simulink library "Batteries"  (R2025b)
settings: Solver=VariableStepAuto  StartTime=0.0  StopTime=10.0  RelTol=1e-3
undefined symbols (not defined in the file or in its folder): battery_builder_rtmsupport, gcbh
libraries: Batteries_lib x12
(part 1 of 2)
settings Model: Creator=Ashwin VJ  LastModifiedBy=Ashwin VJ

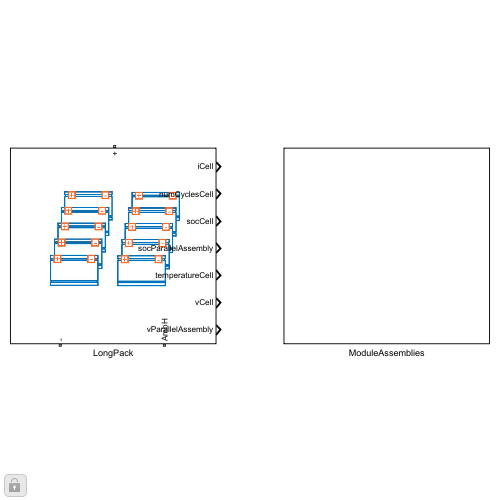
[thumbnail: Simulink's stored preview of the top-level diagram]
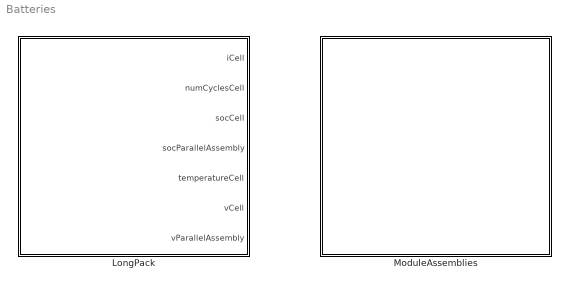
== system Batteries ==
  LongPack : Subsystem  LoadFcn=battery_builder_rtmsupport('loadfcn',gcbh);
      settings: CopyFcn=battery_builder_rtmsupport('copyfcn',gcbh);  PreCopyFcn=battery_builder_rtmsupport('precopyfcn',gcbh);  PreDeleteFcn=battery_builder_rtmsupport('predeletefcn',gcbh);  PortSchema="{\"entries\":[{\"content\":{\"sides\":[{\"content\":{\"connectorIds\":[\"LConn1\"]},\"type\":\"ConnectorPlacement.EquallySpacedRectSide\",\"uuid\":\"4fe37960-74fc-413e-9859-48e6f871084a\"},{\"content\":{\"connectorIds\":[\"RConn1\",\"RConn2\"],\"side\":\"RIGHT\"},\"type\":\"ConnectorPlacement.EquallySpacedRectSide\",\"uuid\":\"59d8cb7e-b3c6-46ea-9337-4df7c2d713cd\"},{\"content\":{\"side\":\"TOP\"},\"type\":\"ConnectorPlacement.EquallySpacedRectSide\",\"uuid\":\"862fb2f6-2715-4d64-bb2a-a0e059187e75\"},{\"content\":{\"connectorIds\":[\"Out1\",\"Out2\",\"Out3\",\"Out4\",\"Out5\",\"Out6\",\"Out7\"],\"side\":\"BOTTOM\"},\"type\":\"ConnectorPlacement.EquallySpacedRectSide\",\"uuid\":\"1041eb17-222a-4b12-b771-3ff8ff1e176b\"}]},\"type\":\"ConnectorPlacement.EquallySpacedConnector\",\"uuid\":\"a86749cc-7dd3-46dc-b06c-c30e9499a85b\"}],\"packageUris\":[\"http://schema.mathworks.com/mf0/Connector/R2020b\"],\"version\":\"1.0\"}"
      mask Display: image('$imagefile')
  ModuleAssemblies : Subsystem

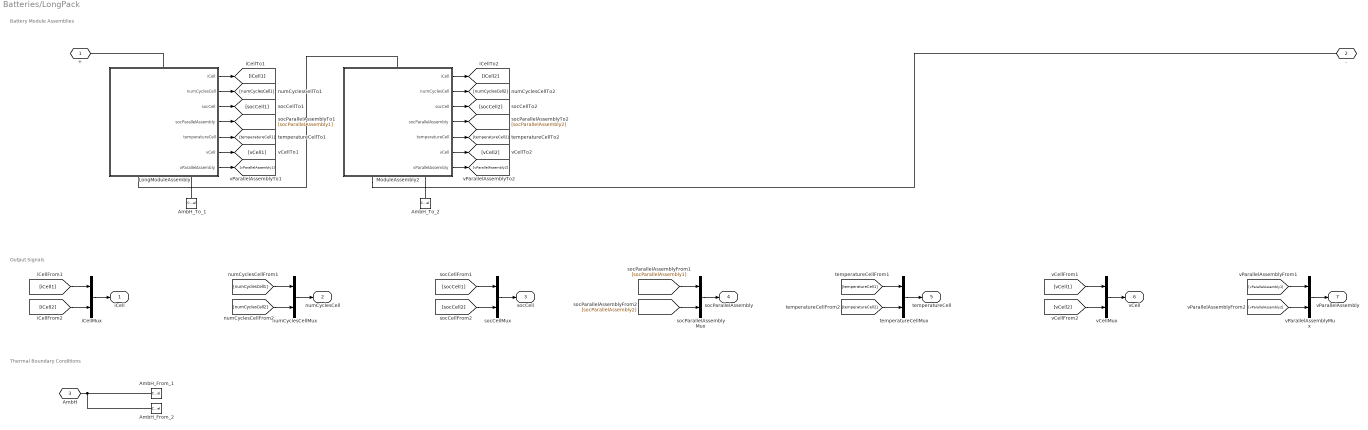
== system Batteries/LongPack ==
  note: Battery Module Assemblies
  note: Output Signals
  note: Thermal Boundary Conditions
  AmbH_From_1 : ConnectionLabel  Label=ambH_1
  AmbH_From_2 : ConnectionLabel  Label=ambH_2
  AmbH_To_1 : ConnectionLabel  Label=ambH_1
  AmbH_To_2 : ConnectionLabel  Label=ambH_2
  LongModuleAssembly : Subsystem  LoadFcn=battery_builder_rtmsupport('loadfcn',gcbh);
      settings: CopyFcn=battery_builder_rtmsupport('copyfcn',gcbh);  PreCopyFcn=battery_builder_rtmsupport('precopyfcn',gcbh);  PreDeleteFcn=battery_builder_rtmsupport('predeletefcn',gcbh);  PortSchema="{\"entries\":[{\"content\":{\"sides\":[{\"content\":{\"connectorIds\":[\"LConn1\"]},\"type\":\"ConnectorPlacement.EquallySpacedRectSide\",\"uuid\":\"4fe37960-74fc-413e-9859-48e6f871084a\"},{\"content\":{\"connectorIds\":[\"RConn1\",\"RConn2\"],\"side\":\"RIGHT\"},\"type\":\"ConnectorPlacement.EquallySpacedRectSide\",\"uuid\":\"59d8cb7e-b3c6-46ea-9337-4df7c2d713cd\"},{\"content\":{\"side\":\"TOP\"},\"type\":\"ConnectorPlacement.EquallySpacedRectSide\",\"uuid\":\"862fb2f6-2715-4d64-bb2a-a0e059187e75\"},{\"content\":{\"connectorIds\":[\"Out1\",\"Out2\",\"Out3\",\"Out4\",\"Out5\",\"Out6\",\"Out7\"],\"side\":\"BOTTOM\"},\"type\":\"ConnectorPlacement.EquallySpacedRectSide\",\"uuid\":\"c7371d3c-3698-4067-a274-1cbefaf9f93a\"}]},\"type\":\"ConnectorPlacement.EquallySpacedConnector\",\"uuid\":\"a86749cc-7dd3-46dc-b06c-c30e9499a85b\"}],\"packageUris\":[\"http://schema.mathworks.com/mf0/Connector/R2020b\"],\"version\":\"1.0\"}"
      mask Display: image('$imagefile')
  ModuleAssembly2 : Subsystem  LoadFcn=battery_builder_rtmsupport('loadfcn',gcbh);
      settings: CopyFcn=battery_builder_rtmsupport('copyfcn',gcbh);  PreCopyFcn=battery_builder_rtmsupport('precopyfcn',gcbh);  PreDeleteFcn=battery_builder_rtmsupport('predeletefcn',gcbh);  PortSchema="{\"entries\":[{\"content\":{\"sides\":[{\"content\":{\"connectorIds\":[\"LConn1\"]},\"type\":\"ConnectorPlacement.EquallySpacedRectSide\",\"uuid\":\"4fe37960-74fc-413e-9859-48e6f871084a\"},{\"content\":{\"connectorIds\":[\"RConn1\",\"RConn2\"],\"side\":\"RIGHT\"},\"type\":\"ConnectorPlacement.EquallySpacedRectSide\",\"uuid\":\"59d8cb7e-b3c6-46ea-9337-4df7c2d713cd\"},{\"content\":{\"side\":\"TOP\"},\"type\":\"ConnectorPlacement.EquallySpacedRectSide\",\"uuid\":\"862fb2f6-2715-4d64-bb2a-a0e059187e75\"},{\"content\":{\"connectorIds\":[\"Out1\",\"Out2\",\"Out3\",\"Out4\",\"Out5\",\"Out6\",\"Out7\"],\"side\":\"BOTTOM\"},\"type\":\"ConnectorPlacement.EquallySpacedRectSide\",\"uuid\":\"c7371d3c-3698-4067-a274-1cbefaf9f93a\"}]},\"type\":\"ConnectorPlacement.EquallySpacedConnector\",\"uuid\":\"a86749cc-7dd3-46dc-b06c-c30e9499a85b\"}],\"packageUris\":[\"http://schema.mathworks.com/mf0/Connector/R2020b\"],\"version\":\"1.0\"}"
      mask Display: image('$imagefile')
  iCellMux : Mux  Inputs=2
  numCyclesCellMux : Mux  Inputs=2
  socCellMux : Mux  Inputs=2
  socParallelAssemblyMux : Mux  Inputs=2
  temperatureCellMux : Mux  Inputs=2
  vCellMux : Mux  Inputs=2
  vParallelAssemblyMux : Mux  Inputs=2
  + : PMIOPort  Side=Left
  - : PMIOPort  Port=2  Side=Right
  AmbH : PMIOPort  Port=3  Side=Right  ConnectionType=Connection: foundation.thermal.thermal
  iCell : Outport
  numCyclesCell : Outport  Port=2
  socCell : Outport  Port=3
  socParallelAssembly : Outport  Port=4
  temperatureCell : Outport  Port=5
  vCell : Outport  Port=6
  vParallelAssembly : Outport  Port=7
  wires:
  LongModuleAssembly/1(iCell) -> [iCell1]
  iCellMux/1 -> iCell/1
  [iCell1] -> iCellMux/1
  LongModuleAssembly/2(numCyclesCell) -> [numCyclesCell1]
  numCyclesCellMux/1 -> numCyclesCell/1
  [numCyclesCell1] -> numCyclesCellMux/1
  LongModuleAssembly/3(socCell) -> [socCell1]
  socCellMux/1 -> socCell/1
  [socCell1] -> socCellMux/1
  LongModuleAssembly/4(socParallelAssembly) -> [socParallelAssembly1]
  socParallelAssemblyMux/1 -> socParallelAssembly/1
  [socParallelAssembly1] -> socParallelAssemblyMux/1
  LongModuleAssembly/5(temperatureCell) -> [temperatureCell1]
  temperatureCellMux/1 -> temperatureCell/1
  [temperatureCell1] -> temperatureCellMux/1
  LongModuleAssembly/6(vCell) -> [vCell1]
  vCellMux/1 -> vCell/1
  [vCell1] -> vCellMux/1
  LongModuleAssembly/7(vParallelAssembly) -> [vParallelAssembly1]
  vParallelAssemblyMux/1 -> vParallelAssembly/1
  [vParallelAssembly1] -> vParallelAssemblyMux/1
  ModuleAssembly2/1(iCell) -> [iCell2]
  [iCell2] -> iCellMux/2
  ModuleAssembly2/2(numCyclesCell) -> [numCyclesCell2]
  [numCyclesCell2] -> numCyclesCellMux/2
  ModuleAssembly2/3(socCell) -> [socCell2]
  [socCell2] -> socCellMux/2
  ModuleAssembly2/4(socParallelAssembly) -> [socParallelAssembly2]
  [socParallelAssembly2] -> socParallelAssemblyMux/2
  ModuleAssembly2/5(temperatureCell) -> [temperatureCell2]
  [temperatureCell2] -> temperatureCellMux/2
  ModuleAssembly2/6(vCell) -> [vCell2]
  [vCell2] -> vCellMux/2
  ModuleAssembly2/7(vParallelAssembly) -> [vParallelAssembly2]
  [vParallelAssembly2] -> vParallelAssemblyMux/2
  connections:
  ModuleAssembly2/LConn1 -- LongModuleAssembly/RConn1
  LongModuleAssembly/LConn1 -- +/RConn1
  ModuleAssembly2/RConn1 -- -/RConn1
  AmbH_To_1/LConn1 -- LongModuleAssembly/RConn2
  AmbH/RConn1 -- AmbH_From_1/LConn1 -- AmbH_From_2/LConn1
  AmbH_To_2/LConn1 -- ModuleAssembly2/RConn2

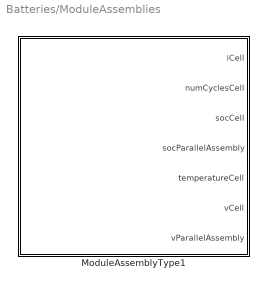
== system Batteries/ModuleAssemblies ==
  ModuleAssemblyType1 : Subsystem  LoadFcn=battery_builder_rtmsupport('loadfcn',gcbh);
      settings: CopyFcn=battery_builder_rtmsupport('copyfcn',gcbh);  PreCopyFcn=battery_builder_rtmsupport('precopyfcn',gcbh);  PreDeleteFcn=battery_builder_rtmsupport('predeletefcn',gcbh);  PortSchema="{\"entries\":[{\"content\":{\"sides\":[{\"content\":{\"connectorIds\":[\"LConn1\"]},\"type\":\"ConnectorPlacement.EquallySpacedRectSide\",\"uuid\":\"4fe37960-74fc-413e-9859-48e6f871084a\"},{\"content\":{\"connectorIds\":[\"RConn1\",\"RConn2\"],\"side\":\"RIGHT\"},\"type\":\"ConnectorPlacement.EquallySpacedRectSide\",\"uuid\":\"59d8cb7e-b3c6-46ea-9337-4df7c2d713cd\"},{\"content\":{\"side\":\"TOP\"},\"type\":\"ConnectorPlacement.EquallySpacedRectSide\",\"uuid\":\"862fb2f6-2715-4d64-bb2a-a0e059187e75\"},{\"content\":{\"connectorIds\":[\"Out1\",\"Out2\",\"Out3\",\"Out4\",\"Out5\",\"Out6\",\"Out7\"],\"side\":\"BOTTOM\"},\"type\":\"ConnectorPlacement.EquallySpacedRectSide\",\"uuid\":\"c7371d3c-3698-4067-a274-1cbefaf9f93a\"}]},\"type\":\"ConnectorPlacement.EquallySpacedConnector\",\"uuid\":\"a86749cc-7dd3-46dc-b06c-c30e9499a85b\"}],\"packageUris\":[\"http://schema.mathworks.com/mf0/Connector/R2020b\"],\"version\":\"1.0\"}"
      mask Display: image('$imagefile')

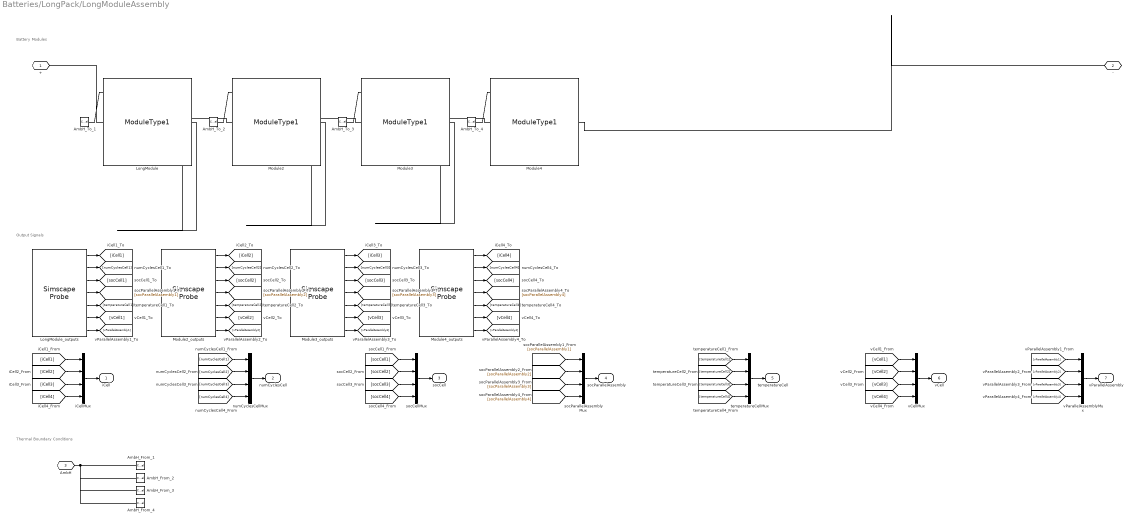
== system Batteries/LongPack/LongModuleAssembly ==
  note: Thermal Boundary Conditions
  note: Output Signals
  note: Battery Modules
  AmbH_From_1 : ConnectionLabel  Label=ambH_1
  AmbH_From_2 : ConnectionLabel  Label=ambH_2
  AmbH_From_3 : ConnectionLabel  Label=ambH_3
  AmbH_From_4 : ConnectionLabel  Label=ambH_4
  AmbH_To_1 : ConnectionLabel  Label=ambH_1
  AmbH_To_2 : ConnectionLabel  Label=ambH_2
  AmbH_To_3 : ConnectionLabel  Label=ambH_3
  AmbH_To_4 : ConnectionLabel  Label=ambH_4
  LongModule : Batteries_lib/Modules/ModuleType1  SOC_vecCell=[0, .1, .25, .5, .75, .9, 1]  T_vecCell=[278, 293, 313] K  V0_matCell=[3.49, 3.5, 3.51; 3.55, 3.57, 3.56; 3.62, 3.63, 3.64; 3.71, 3.71, 3.72; 3.91, 3.93, 3.94; 4.07, 4.08, 4.08; 4.19, 4.19, 4.19] V  V_rangeCell=[0, inf] V  R0_matCell=[.0117, .0085, .009; .011, .0085, .009; .0114, .0087, .0092; .0107, .0082, .0088; .0107, .0083, .0091; .0113, .0085, .0089; .0116, .0085, .0089] Ohm  AHCell=27 A*hr  extrapolation_optionCell=simscape.enum.extrapolation.nearest  thermal_massCell=100 J/K  CoolantResistance=1.2 K/W  AmbientResistance=25 K/W  P=20  S=2  iCell_specify=off  iCell_priority=None  iCell=0 A  iCell_nominal_specify=off  iCell_nominal_value=1  iCell_nominal_unit=A  vCell_specify=off  vCell_priority=None  vCell=0 V  vCell_nominal_specify=off  vCell_nominal_value=1  vCell_nominal_unit=V  socCell_specify=off  socCell_priority=High  socCell=1  socCell_nominal_specify=off  socCell_nominal_value=1  socCell_nominal_unit=1  numCyclesCell_specify=off  numCyclesCell_priority=High  numCyclesCell=0  numCyclesCell_nominal_specify=off  numCyclesCell_nominal_value=1  numCyclesCell_nominal_unit=1  temperatureCell_specify=off  temperatureCell_priority=High  temperatureCell=298.15 K  temperatureCell_nominal_specify=off  temperatureCell_nominal_value=1  temperatureCell_nominal_unit=K  vParallelAssembly_specify=off  vParallelAssembly_priority=None  vParallelAssembly=repmat(0, 2, 1) V  vParallelAssembly_nominal_specify=off  vParallelAssembly_nominal_value=1  vParallelAssembly_nominal_unit=V  socParallelAssembly_specify=off  socParallelAssembly_priority=None  socParallelAssembly=repmat(1, 2, 1)  socParallelAssembly_nominal_specify=off  socParallelAssembly_nominal_value=1  socParallelAssembly_nominal_unit=1
      settings: InternalSimscapePortConfiguration="{\"Bottom\":[{\"id\":\"n\",\"label\":\"-\",\"type\":\"foundation.electrical.electrical\"}],\"Left\":[{\"id\":\"AmbH\",\"label\":\"AmbH\",\"type\":\"foundation.thermal.thermal\"}],\"Right\":[],\"Top\":[{\"id\":\"p\",\"label\":\"+\",\"type\":\"foundation.electrical.electrical\"},{\"id\":\"TopExtClnt\",\"label\":\"CPT\",\"type\":\"foundation.thermal.thermal\"}]}"
  LongModule_outputs : SimscapeProbe  BoundBlock=105  Variables="{\"iCell\":{\"Probing\":\"ON\"},\"numCyclesCell\":{\"Probing\":\"ON\"},\"socCell\":{\"Probing\":\"ON\"},\"socParallelAssembly\":{\"Probing\":\"ON\"},\"temperatureCell\":{\"Probing\":\"ON\"},\"vCell\":{\"Probing\":\"ON\"},\"vParallelAssembly\":{\"Probing\":\"ON\"}}"
  Module2 : Batteries_lib/Modules/ModuleType1  SOC_vecCell=[0, .1, .25, .5, .75, .9, 1]  T_vecCell=[278, 293, 313] K  V0_matCell=[3.49, 3.5, 3.51; 3.55, 3.57, 3.56; 3.62, 3.63, 3.64; 3.71, 3.71, 3.72; 3.91, 3.93, 3.94; 4.07, 4.08, 4.08; 4.19, 4.19, 4.19] V  V_rangeCell=[0, inf] V  R0_matCell=[.0117, .0085, .009; .011, .0085, .009; .0114, .0087, .0092; .0107, .0082, .0088; .0107, .0083, .0091; .0113, .0085, .0089; .0116, .0085, .0089] Ohm  AHCell=27 A*hr  extrapolation_optionCell=simscape.enum.extrapolation.nearest  thermal_massCell=100 J/K  CoolantResistance=1.2 K/W  AmbientResistance=25 K/W  P=20  S=2  iCell_specify=off  iCell_priority=None  iCell=0 A  iCell_nominal_specify=off  iCell_nominal_value=1  iCell_nominal_unit=A  vCell_specify=off  vCell_priority=None  vCell=0 V  vCell_nominal_specify=off  vCell_nominal_value=1  vCell_nominal_unit=V  socCell_specify=off  socCell_priority=High  socCell=1  socCell_nominal_specify=off  socCell_nominal_value=1  socCell_nominal_unit=1  numCyclesCell_specify=off  numCyclesCell_priority=High  numCyclesCell=0  numCyclesCell_nominal_specify=off  numCyclesCell_nominal_value=1  numCyclesCell_nominal_unit=1  temperatureCell_specify=off  temperatureCell_priority=High  temperatureCell=298.15 K  temperatureCell_nominal_specify=off  temperatureCell_nominal_value=1  temperatureCell_nominal_unit=K  vParallelAssembly_specify=off  vParallelAssembly_priority=None  vParallelAssembly=repmat(0, 2, 1) V  vParallelAssembly_nominal_specify=off  vParallelAssembly_nominal_value=1  vParallelAssembly_nominal_unit=V  socParallelAssembly_specify=off  socParallelAssembly_priority=None  socParallelAssembly=repmat(1, 2, 1)  socParallelAssembly_nominal_specify=off  socParallelAssembly_nominal_value=1  socParallelAssembly_nominal_unit=1
      settings: InternalSimscapePortConfiguration="{\"Bottom\":[{\"id\":\"n\",\"label\":\"-\",\"type\":\"foundation.electrical.electrical\"}],\"Left\":[{\"id\":\"AmbH\",\"label\":\"AmbH\",\"type\":\"foundation.thermal.thermal\"}],\"Right\":[],\"Top\":[{\"id\":\"p\",\"label\":\"+\",\"type\":\"foundation.electrical.electrical\"},{\"id\":\"TopExtClnt\",\"label\":\"CPT\",\"type\":\"foundation.thermal.thermal\"}]}"
  Module2_outputs : SimscapeProbe  BoundBlock=107  Variables="{\"iCell\":{\"Probing\":\"ON\"},\"numCyclesCell\":{\"Probing\":\"ON\"},\"socCell\":{\"Probing\":\"ON\"},\"socParallelAssembly\":{\"Probing\":\"ON\"},\"temperatureCell\":{\"Probing\":\"ON\"},\"vCell\":{\"Probing\":\"ON\"},\"vParallelAssembly\":{\"Probing\":\"ON\"}}"
  Module3 : Batteries_lib/Modules/ModuleType1  SOC_vecCell=[0, .1, .25, .5, .75, .9, 1]  T_vecCell=[278, 293, 313] K  V0_matCell=[3.49, 3.5, 3.51; 3.55, 3.57, 3.56; 3.62, 3.63, 3.64; 3.71, 3.71, 3.72; 3.91, 3.93, 3.94; 4.07, 4.08, 4.08; 4.19, 4.19, 4.19] V  V_rangeCell=[0, inf] V  R0_matCell=[.0117, .0085, .009; .011, .0085, .009; .0114, .0087, .0092; .0107, .0082, .0088; .0107, .0083, .0091; .0113, .0085, .0089; .0116, .0085, .0089] Ohm  AHCell=27 A*hr  extrapolation_optionCell=simscape.enum.extrapolation.nearest  thermal_massCell=100 J/K  CoolantResistance=1.2 K/W  AmbientResistance=25 K/W  P=20  S=2  iCell_specify=off  iCell_priority=None  iCell=0 A  iCell_nominal_specify=off  iCell_nominal_value=1  iCell_nominal_unit=A  vCell_specify=off  vCell_priority=None  vCell=0 V  vCell_nominal_specify=off  vCell_nominal_value=1  vCell_nominal_unit=V  socCell_specify=off  socCell_priority=High  socCell=1  socCell_nominal_specify=off  socCell_nominal_value=1  socCell_nominal_unit=1  numCyclesCell_specify=off  numCyclesCell_priority=High  numCyclesCell=0  numCyclesCell_nominal_specify=off  numCyclesCell_nominal_value=1  numCyclesCell_nominal_unit=1  temperatureCell_specify=off  temperatureCell_priority=High  temperatureCell=298.15 K  temperatureCell_nominal_specify=off  temperatureCell_nominal_value=1  temperatureCell_nominal_unit=K  vParallelAssembly_specify=off  vParallelAssembly_priority=None  vParallelAssembly=repmat(0, 2, 1) V  vParallelAssembly_nominal_specify=off  vParallelAssembly_nominal_value=1  vParallelAssembly_nominal_unit=V  socParallelAssembly_specify=off  socParallelAssembly_priority=None  socParallelAssembly=repmat(1, 2, 1)  socParallelAssembly_nominal_specify=off  socParallelAssembly_nominal_value=1  socParallelAssembly_nominal_unit=1
      settings: InternalSimscapePortConfiguration="{\"Bottom\":[{\"id\":\"n\",\"label\":\"-\",\"type\":\"foundation.electrical.electrical\"}],\"Left\":[{\"id\":\"AmbH\",\"label\":\"AmbH\",\"type\":\"foundation.thermal.thermal\"}],\"Right\":[],\"Top\":[{\"id\":\"p\",\"label\":\"+\",\"type\":\"foundation.electrical.electrical\"},{\"id\":\"TopExtClnt\",\"label\":\"CPT\",\"type\":\"foundation.thermal.thermal\"}]}"
  Module3_outputs : SimscapeProbe  BoundBlock=109  Variables="{\"iCell\":{\"Probing\":\"ON\"},\"numCyclesCell\":{\"Probing\":\"ON\"},\"socCell\":{\"Probing\":\"ON\"},\"socParallelAssembly\":{\"Probing\":\"ON\"},\"temperatureCell\":{\"Probing\":\"ON\"},\"vCell\":{\"Probing\":\"ON\"},\"vParallelAssembly\":{\"Probing\":\"ON\"}}"
  Module4 : Batteries_lib/Modules/ModuleType1  SOC_vecCell=[0, .1, .25, .5, .75, .9, 1]  T_vecCell=[278, 293, 313] K  V0_matCell=[3.49, 3.5, 3.51; 3.55, 3.57, 3.56; 3.62, 3.63, 3.64; 3.71, 3.71, 3.72; 3.91, 3.93, 3.94; 4.07, 4.08, 4.08; 4.19, 4.19, 4.19] V  V_rangeCell=[0, inf] V  R0_matCell=[.0117, .0085, .009; .011, .0085, .009; .0114, .0087, .0092; .0107, .0082, .0088; .0107, .0083, .0091; .0113, .0085, .0089; .0116, .0085, .0089] Ohm  AHCell=27 A*hr  extrapolation_optionCell=simscape.enum.extrapolation.nearest  thermal_massCell=100 J/K  CoolantResistance=1.2 K/W  AmbientResistance=25 K/W  P=20  S=2  iCell_specify=off  iCell_priority=None  iCell=0 A  iCell_nominal_specify=off  iCell_nominal_value=1  iCell_nominal_unit=A  vCell_specify=off  vCell_priority=None  vCell=0 V  vCell_nominal_specify=off  vCell_nominal_value=1  vCell_nominal_unit=V  socCell_specify=off  socCell_priority=High  socCell=1  socCell_nominal_specify=off  socCell_nominal_value=1  socCell_nominal_unit=1  numCyclesCell_specify=off  numCyclesCell_priority=High  numCyclesCell=0  numCyclesCell_nominal_specify=off  numCyclesCell_nominal_value=1  numCyclesCell_nominal_unit=1  temperatureCell_specify=off  temperatureCell_priority=High  temperatureCell=298.15 K  temperatureCell_nominal_specify=off  temperatureCell_nominal_value=1  temperatureCell_nominal_unit=K  vParallelAssembly_specify=off  vParallelAssembly_priority=None  vParallelAssembly=repmat(0, 2, 1) V  vParallelAssembly_nominal_specify=off  vParallelAssembly_nominal_value=1  vParallelAssembly_nominal_unit=V  socParallelAssembly_specify=off  socParallelAssembly_priority=None  socParallelAssembly=repmat(1, 2, 1)  socParallelAssembly_nominal_specify=off  socParallelAssembly_nominal_value=1  socParallelAssembly_nominal_unit=1
      settings: InternalSimscapePortConfiguration="{\"Bottom\":[{\"id\":\"n\",\"label\":\"-\",\"type\":\"foundation.electrical.electrical\"}],\"Left\":[{\"id\":\"AmbH\",\"label\":\"AmbH\",\"type\":\"foundation.thermal.thermal\"}],\"Right\":[],\"Top\":[{\"id\":\"p\",\"label\":\"+\",\"type\":\"foundation.electrical.electrical\"},{\"id\":\"TopExtClnt\",\"label\":\"CPT\",\"type\":\"foundation.thermal.thermal\"}]}"
  Module4_outputs : SimscapeProbe  BoundBlock=111  Variables="{\"iCell\":{\"Probing\":\"ON\"},\"numCyclesCell\":{\"Probing\":\"ON\"},\"socCell\":{\"Probing\":\"ON\"},\"socParallelAssembly\":{\"Probing\":\"ON\"},\"temperatureCell\":{\"Probing\":\"ON\"},\"vCell\":{\"Probing\":\"ON\"},\"vParallelAssembly\":{\"Probing\":\"ON\"}}"
  iCellMux : Mux
  numCyclesCellMux : Mux
  socCellMux : Mux
  socParallelAssemblyMux : Mux
  temperatureCellMux : Mux
  vCellMux : Mux
  vParallelAssemblyMux : Mux
  + : PMIOPort  Side=Left
  - : PMIOPort  Port=2  Side=Right
  AmbH : PMIOPort  Port=3  Side=Right  ConnectionType=Connection: foundation.thermal.thermal
  iCell : Outport
  numCyclesCell : Outport  Port=2
  socCell : Outport  Port=3
  socParallelAssembly : Outport  Port=4
  temperatureCell : Outport  Port=5
  vCell : Outport  Port=6
  vParallelAssembly : Outport  Port=7
  wires:
  [vParallelAssembly4] -> vParallelAssemblyMux/4
  Module4_outputs/7 -> [vParallelAssembly4]
  [vCell4] -> vCellMux/4
  Module4_outputs/6 -> [vCell4]
  [temperatureCell4] -> temperatureCellMux/4
  Module4_outputs/5 -> [temperatureCell4]
  [socParallelAssembly4] -> socParallelAssemblyMux/4
  Module4_outputs/4 -> [socParallelAssembly4]
  [socCell4] -> socCellMux/4
  Module4_outputs/3 -> [socCell4]
  [numCyclesCell4] -> numCyclesCellMux/4
  Module4_outputs/2 -> [numCyclesCell4]
  [iCell4] -> iCellMux/4
  Module4_outputs/1 -> [iCell4]
  [vParallelAssembly3] -> vParallelAssemblyMux/3
  Module3_outputs/7 -> [vParallelAssembly3]
  [vCell3] -> vCellMux/3
  Module3_outputs/6 -> [vCell3]
  [temperatureCell3] -> temperatureCellMux/3
  Module3_outputs/5 -> [temperatureCell3]
  [socParallelAssembly3] -> socParallelAssemblyMux/3
  Module3_outputs/4 -> [socParallelAssembly3]
  [socCell3] -> socCellMux/3
  Module3_outputs/3 -> [socCell3]
  [numCyclesCell3] -> numCyclesCellMux/3
  Module3_outputs/2 -> [numCyclesCell3]
  [iCell3] -> iCellMux/3
  Module3_outputs/1 -> [iCell3]
  [vParallelAssembly2] -> vParallelAssemblyMux/2
  Module2_outputs/7 -> [vParallelAssembly2]
  [vCell2] -> vCellMux/2
  Module2_outputs/6 -> [vCell2]
  [temperatureCell2] -> temperatureCellMux/2
  Module2_outputs/5 -> [temperatureCell2]
  [socParallelAssembly2] -> socParallelAssemblyMux/2
  Module2_outputs/4 -> [socParallelAssembly2]
  [socCell2] -> socCellMux/2
  Module2_outputs/3 -> [socCell2]
  [numCyclesCell2] -> numCyclesCellMux/2
  Module2_outputs/2 -> [numCyclesCell2]
  [iCell2] -> iCellMux/2
  Module2_outputs/1 -> [iCell2]
  [vParallelAssembly1] -> vParallelAssemblyMux/1
  vParallelAssemblyMux/1 -> vParallelAssembly/1
  LongModule_outputs/7 -> [vParallelAssembly1]
  [vCell1] -> vCellMux/1
  vCellMux/1 -> vCell/1
  LongModule_outputs/6 -> [vCell1]
  [temperatureCell1] -> temperatureCellMux/1
  temperatureCellMux/1 -> temperatureCell/1
  LongModule_outputs/5 -> [temperatureCell1]
  [socParallelAssembly1] -> socParallelAssemblyMux/1
  socParallelAssemblyMux/1 -> socParallelAssembly/1
  LongModule_outputs/4 -> [socParallelAssembly1]
  [socCell1] -> socCellMux/1
  socCellMux/1 -> socCell/1
  LongModule_outputs/3 -> [socCell1]
  [numCyclesCell1] -> numCyclesCellMux/1
  numCyclesCellMux/1 -> numCyclesCell/1
  LongModule_outputs/2 -> [numCyclesCell1]
  [iCell1] -> iCellMux/1
  iCellMux/1 -> iCell/1
  LongModule_outputs/1 -> [iCell1]
  connections:
  AmbH_To_4/LConn1 -- Module4/LConn1
  AmbH_To_3/LConn1 -- Module3/LConn1
  AmbH_To_2/LConn1 -- Module2/LConn1
  AmbH_From_4/LConn1 -- AmbH/RConn1 -- AmbH_From_3/LConn1 -- AmbH_From_2/LConn1 -- AmbH_From_1/LConn1
  AmbH_To_1/LConn1 -- LongModule/LConn1
  Module4/RConn1 -- -/RConn1
  LongModule/LConn2 -- +/RConn1
  Module4/LConn2 -- Module3/RConn1
  Module3/LConn2 -- Module2/RConn1
  Module2/LConn2 -- LongModule/RConn1

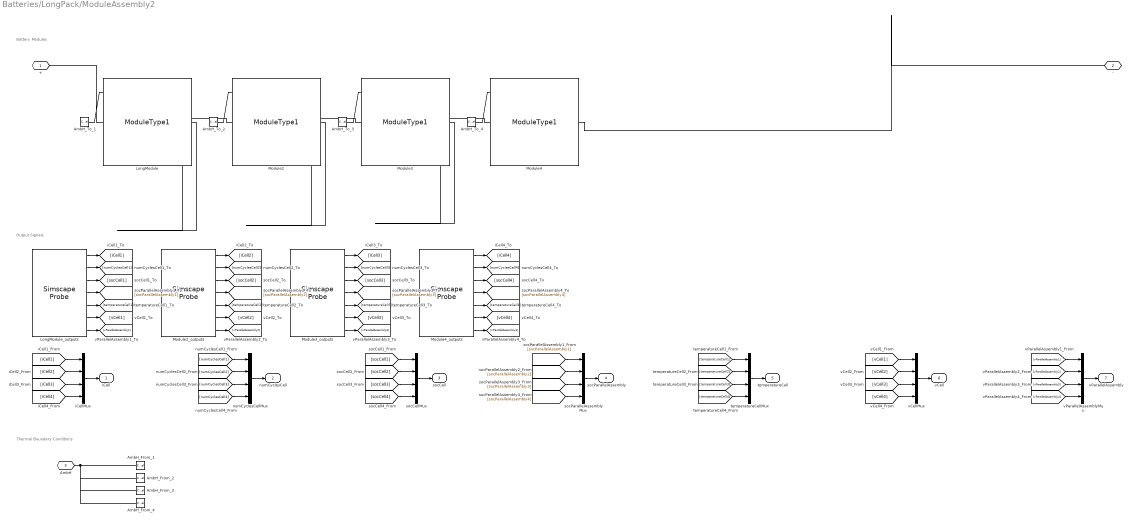
== system Batteries/LongPack/ModuleAssembly2 ==
  note: Thermal Boundary Conditions
  note: Output Signals
  note: Battery Modules
  AmbH_From_1 : ConnectionLabel  Label=ambH_1
  AmbH_From_2 : ConnectionLabel  Label=ambH_2
  AmbH_From_3 : ConnectionLabel  Label=ambH_3
  AmbH_From_4 : ConnectionLabel  Label=ambH_4
  AmbH_To_1 : ConnectionLabel  Label=ambH_1
  AmbH_To_2 : ConnectionLabel  Label=ambH_2
  AmbH_To_3 : ConnectionLabel  Label=ambH_3
  AmbH_To_4 : ConnectionLabel  Label=ambH_4
  LongModule : Batteries_lib/Modules/ModuleType1  SOC_vecCell=[0, .1, .25, .5, .75, .9, 1]  T_vecCell=[278, 293, 313] K  V0_matCell=[3.49, 3.5, 3.51; 3.55, 3.57, 3.56; 3.62, 3.63, 3.64; 3.71, 3.71, 3.72; 3.91, 3.93, 3.94; 4.07, 4.08, 4.08; 4.19, 4.19, 4.19] V  V_rangeCell=[0, inf] V  R0_matCell=[.0117, .0085, .009; .011, .0085, .009; .0114, .0087, .0092; .0107, .0082, .0088; .0107, .0083, .0091; .0113, .0085, .0089; .0116, .0085, .0089] Ohm  AHCell=27 A*hr  extrapolation_optionCell=simscape.enum.extrapolation.nearest  thermal_massCell=100 J/K  CoolantResistance=1.2 K/W  AmbientResistance=25 K/W  P=20  S=2  iCell_specify=off  iCell_priority=None  iCell=0 A  iCell_nominal_specify=off  iCell_nominal_value=1  iCell_nominal_unit=A  vCell_specify=off  vCell_priority=None  vCell=0 V  vCell_nominal_specify=off  vCell_nominal_value=1  vCell_nominal_unit=V  socCell_specify=off  socCell_priority=High  socCell=1  socCell_nominal_specify=off  socCell_nominal_value=1  socCell_nominal_unit=1  numCyclesCell_specify=off  numCyclesCell_priority=High  numCyclesCell=0  numCyclesCell_nominal_specify=off  numCyclesCell_nominal_value=1  numCyclesCell_nominal_unit=1  temperatureCell_specify=off  temperatureCell_priority=High  temperatureCell=298.15 K  temperatureCell_nominal_specify=off  temperatureCell_nominal_value=1  temperatureCell_nominal_unit=K  vParallelAssembly_specify=off  vParallelAssembly_priority=None  vParallelAssembly=repmat(0, 2, 1) V  vParallelAssembly_nominal_specify=off  vParallelAssembly_nominal_value=1  vParallelAssembly_nominal_unit=V  socParallelAssembly_specify=off  socParallelAssembly_priority=None  socParallelAssembly=repmat(1, 2, 1)  socParallelAssembly_nominal_specify=off  socParallelAssembly_nominal_value=1  socParallelAssembly_nominal_unit=1
      settings: InternalSimscapePortConfiguration="{\"Bottom\":[{\"id\":\"n\",\"label\":\"-\",\"type\":\"foundation.electrical.electrical\"}],\"Left\":[{\"id\":\"AmbH\",\"label\":\"AmbH\",\"type\":\"foundation.thermal.thermal\"}],\"Right\":[],\"Top\":[{\"id\":\"p\",\"label\":\"+\",\"type\":\"foundation.electrical.electrical\"},{\"id\":\"TopExtClnt\",\"label\":\"CPT\",\"type\":\"foundation.thermal.thermal\"}]}"
  LongModule_outputs : SimscapeProbe  BoundBlock=198  Variables="{\"iCell\":{\"Probing\":\"ON\"},\"numCyclesCell\":{\"Probing\":\"ON\"},\"socCell\":{\"Probing\":\"ON\"},\"socParallelAssembly\":{\"Probing\":\"ON\"},\"temperatureCell\":{\"Probing\":\"ON\"},\"vCell\":{\"Probing\":\"ON\"},\"vParallelAssembly\":{\"Probing\":\"ON\"}}"
  Module2 : Batteries_lib/Modules/ModuleType1  SOC_vecCell=[0, .1, .25, .5, .75, .9, 1]  T_vecCell=[278, 293, 313] K  V0_matCell=[3.49, 3.5, 3.51; 3.55, 3.57, 3.56; 3.62, 3.63, 3.64; 3.71, 3.71, 3.72; 3.91, 3.93, 3.94; 4.07, 4.08, 4.08; 4.19, 4.19, 4.19] V  V_rangeCell=[0, inf] V  R0_matCell=[.0117, .0085, .009; .011, .0085, .009; .0114, .0087, .0092; .0107, .0082, .0088; .0107, .0083, .0091; .0113, .0085, .0089; .0116, .0085, .0089] Ohm  AHCell=27 A*hr  extrapolation_optionCell=simscape.enum.extrapolation.nearest  thermal_massCell=100 J/K  CoolantResistance=1.2 K/W  AmbientResistance=25 K/W  P=20  S=2  iCell_specify=off  iCell_priority=None  iCell=0 A  iCell_nominal_specify=off  iCell_nominal_value=1  iCell_nominal_unit=A  vCell_specify=off  vCell_priority=None  vCell=0 V  vCell_nominal_specify=off  vCell_nominal_value=1  vCell_nominal_unit=V  socCell_specify=off  socCell_priority=High  socCell=1  socCell_nominal_specify=off  socCell_nominal_value=1  socCell_nominal_unit=1  numCyclesCell_specify=off  numCyclesCell_priority=High  numCyclesCell=0  numCyclesCell_nominal_specify=off  numCyclesCell_nominal_value=1  numCyclesCell_nominal_unit=1  temperatureCell_specify=off  temperatureCell_priority=High  temperatureCell=298.15 K  temperatureCell_nominal_specify=off  temperatureCell_nominal_value=1  temperatureCell_nominal_unit=K  vParallelAssembly_specify=off  vParallelAssembly_priority=None  vParallelAssembly=repmat(0, 2, 1) V  vParallelAssembly_nominal_specify=off  vParallelAssembly_nominal_value=1  vParallelAssembly_nominal_unit=V  socParallelAssembly_specify=off  socParallelAssembly_priority=None  socParallelAssembly=repmat(1, 2, 1)  socParallelAssembly_nominal_specify=off  socParallelAssembly_nominal_value=1  socParallelAssembly_nominal_unit=1
      settings: InternalSimscapePortConfiguration="{\"Bottom\":[{\"id\":\"n\",\"label\":\"-\",\"type\":\"foundation.electrical.electrical\"}],\"Left\":[{\"id\":\"AmbH\",\"label\":\"AmbH\",\"type\":\"foundation.thermal.thermal\"}],\"Right\":[],\"Top\":[{\"id\":\"p\",\"label\":\"+\",\"type\":\"foundation.electrical.electrical\"},{\"id\":\"TopExtClnt\",\"label\":\"CPT\",\"type\":\"foundation.thermal.thermal\"}]}"
  Module2_outputs : SimscapeProbe  BoundBlock=200  Variables="{\"iCell\":{\"Probing\":\"ON\"},\"numCyclesCell\":{\"Probing\":\"ON\"},\"socCell\":{\"Probing\":\"ON\"},\"socParallelAssembly\":{\"Probing\":\"ON\"},\"temperatureCell\":{\"Probing\":\"ON\"},\"vCell\":{\"Probing\":\"ON\"},\"vParallelAssembly\":{\"Probing\":\"ON\"}}"
  Module3 : Batteries_lib/Modules/ModuleType1  SOC_vecCell=[0, .1, .25, .5, .75, .9, 1]  T_vecCell=[278, 293, 313] K  V0_matCell=[3.49, 3.5, 3.51; 3.55, 3.57, 3.56; 3.62, 3.63, 3.64; 3.71, 3.71, 3.72; 3.91, 3.93, 3.94; 4.07, 4.08, 4.08; 4.19, 4.19, 4.19] V  V_rangeCell=[0, inf] V  R0_matCell=[.0117, .0085, .009; .011, .0085, .009; .0114, .0087, .0092; .0107, .0082, .0088; .0107, .0083, .0091; .0113, .0085, .0089; .0116, .0085, .0089] Ohm  AHCell=27 A*hr  extrapolation_optionCell=simscape.enum.extrapolation.nearest  thermal_massCell=100 J/K  CoolantResistance=1.2 K/W  AmbientResistance=25 K/W  P=20  S=2  iCell_specify=off  iCell_priority=None  iCell=0 A  iCell_nominal_specify=off  iCell_nominal_value=1  iCell_nominal_unit=A  vCell_specify=off  vCell_priority=None  vCell=0 V  vCell_nominal_specify=off  vCell_nominal_value=1  vCell_nominal_unit=V  socCell_specify=off  socCell_priority=High  socCell=1  socCell_nominal_specify=off  socCell_nominal_value=1  socCell_nominal_unit=1  numCyclesCell_specify=off  numCyclesCell_priority=High  numCyclesCell=0  numCyclesCell_nominal_specify=off  numCyclesCell_nominal_value=1  numCyclesCell_nominal_unit=1  temperatureCell_specify=off  temperatureCell_priority=High  temperatureCell=298.15 K  temperatureCell_nominal_specify=off  temperatureCell_nominal_value=1  temperatureCell_nominal_unit=K  vParallelAssembly_specify=off  vParallelAssembly_priority=None  vParallelAssembly=repmat(0, 2, 1) V  vParallelAssembly_nominal_specify=off  vParallelAssembly_nominal_value=1  vParallelAssembly_nominal_unit=V  socParallelAssembly_specify=off  socParallelAssembly_priority=None  socParallelAssembly=repmat(1, 2, 1)  socParallelAssembly_nominal_specify=off  socParallelAssembly_nominal_value=1  socParallelAssembly_nominal_unit=1
      settings: InternalSimscapePortConfiguration="{\"Bottom\":[{\"id\":\"n\",\"label\":\"-\",\"type\":\"foundation.electrical.electrical\"}],\"Left\":[{\"id\":\"AmbH\",\"label\":\"AmbH\",\"type\":\"foundation.thermal.thermal\"}],\"Right\":[],\"Top\":[{\"id\":\"p\",\"label\":\"+\",\"type\":\"foundation.electrical.electrical\"},{\"id\":\"TopExtClnt\",\"label\":\"CPT\",\"type\":\"foundation.thermal.thermal\"}]}"
  Module3_outputs : SimscapeProbe  BoundBlock=202  Variables="{\"iCell\":{\"Probing\":\"ON\"},\"numCyclesCell\":{\"Probing\":\"ON\"},\"socCell\":{\"Probing\":\"ON\"},\"socParallelAssembly\":{\"Probing\":\"ON\"},\"temperatureCell\":{\"Probing\":\"ON\"},\"vCell\":{\"Probing\":\"ON\"},\"vParallelAssembly\":{\"Probing\":\"ON\"}}"
  Module4 : Batteries_lib/Modules/ModuleType1  SOC_vecCell=[0, .1, .25, .5, .75, .9, 1]  T_vecCell=[278, 293, 313] K  V0_matCell=[3.49, 3.5, 3.51; 3.55, 3.57, 3.56; 3.62, 3.63, 3.64; 3.71, 3.71, 3.72; 3.91, 3.93, 3.94; 4.07, 4.08, 4.08; 4.19, 4.19, 4.19] V  V_rangeCell=[0, inf] V  R0_matCell=[.0117, .0085, .009; .011, .0085, .009; .0114, .0087, .0092; .0107, .0082, .0088; .0107, .0083, .0091; .0113, .0085, .0089; .0116, .0085, .0089] Ohm  AHCell=27 A*hr  extrapolation_optionCell=simscape.enum.extrapolation.nearest  thermal_massCell=100 J/K  CoolantResistance=1.2 K/W  AmbientResistance=25 K/W  P=20  S=2  iCell_specify=off  iCell_priority=None  iCell=0 A  iCell_nominal_specify=off  iCell_nominal_value=1  iCell_nominal_unit=A  vCell_specify=off  vCell_priority=None  vCell=0 V  vCell_nominal_specify=off  vCell_nominal_value=1  vCell_nominal_unit=V  socCell_specify=off  socCell_priority=High  socCell=1  socCell_nominal_specify=off  socCell_nominal_value=1  socCell_nominal_unit=1  numCyclesCell_specify=off  numCyclesCell_priority=High  numCyclesCell=0  numCyclesCell_nominal_specify=off  numCyclesCell_nominal_value=1  numCyclesCell_nominal_unit=1  temperatureCell_specify=off  temperatureCell_priority=High  temperatureCell=298.15 K  temperatureCell_nominal_specify=off  temperatureCell_nominal_value=1  temperatureCell_nominal_unit=K  vParallelAssembly_specify=off  vParallelAssembly_priority=None  vParallelAssembly=repmat(0, 2, 1) V  vParallelAssembly_nominal_specify=off  vParallelAssembly_nominal_value=1  vParallelAssembly_nominal_unit=V  socParallelAssembly_specify=off  socParallelAssembly_priority=None  socParallelAssembly=repmat(1, 2, 1)  socParallelAssembly_nominal_specify=off  socParallelAssembly_nominal_value=1  socParallelAssembly_nominal_unit=1
      settings: InternalSimscapePortConfiguration="{\"Bottom\":[{\"id\":\"n\",\"label\":\"-\",\"type\":\"foundation.electrical.electrical\"}],\"Left\":[{\"id\":\"AmbH\",\"label\":\"AmbH\",\"type\":\"foundation.thermal.thermal\"}],\"Right\":[],\"Top\":[{\"id\":\"p\",\"label\":\"+\",\"type\":\"foundation.electrical.electrical\"},{\"id\":\"TopExtClnt\",\"label\":\"CPT\",\"type\":\"foundation.thermal.thermal\"}]}"
  Module4_outputs : SimscapeProbe  BoundBlock=204  Variables="{\"iCell\":{\"Probing\":\"ON\"},\"numCyclesCell\":{\"Probing\":\"ON\"},\"socCell\":{\"Probing\":\"ON\"},\"socParallelAssembly\":{\"Probing\":\"ON\"},\"temperatureCell\":{\"Probing\":\"ON\"},\"vCell\":{\"Probing\":\"ON\"},\"vParallelAssembly\":{\"Probing\":\"ON\"}}"
  iCellMux : Mux
  numCyclesCellMux : Mux
  socCellMux : Mux
  socParallelAssemblyMux : Mux
  temperatureCellMux : Mux
  vCellMux : Mux
  vParallelAssemblyMux : Mux
  + : PMIOPort  Side=Left
  - : PMIOPort  Port=2  Side=Right
  AmbH : PMIOPort  Port=3  Side=Right  ConnectionType=Connection: foundation.thermal.thermal
  iCell : Outport
  numCyclesCell : Outport  Port=2
  socCell : Outport  Port=3
  socParallelAssembly : Outport  Port=4
  temperatureCell : Outport  Port=5
  vCell : Outport  Port=6
  vParallelAssembly : Outport  Port=7
  wires:
  [vParallelAssembly4] -> vParallelAssemblyMux/4
  Module4_outputs/7 -> [vParallelAssembly4]
  [vCell4] -> vCellMux/4
  Module4_outputs/6 -> [vCell4]
  [temperatureCell4] -> temperatureCellMux/4
  Module4_outputs/5 -> [temperatureCell4]
  [socParallelAssembly4] -> socParallelAssemblyMux/4
  Module4_outputs/4 -> [socParallelAssembly4]
  [socCell4] -> socCellMux/4
  Module4_outputs/3 -> [socCell4]
  [numCyclesCell4] -> numCyclesCellMux/4
  Module4_outputs/2 -> [numCyclesCell4]
  [iCell4] -> iCellMux/4
  Module4_outputs/1 -> [iCell4]
  [vParallelAssembly3] -> vParallelAssemblyMux/3
  Module3_outputs/7 -> [vParallelAssembly3]
  [vCell3] -> vCellMux/3
  Module3_outputs/6 -> [vCell3]
  [temperatureCell3] -> temperatureCellMux/3
  Module3_outputs/5 -> [temperatureCell3]
  [socParallelAssembly3] -> socParallelAssemblyMux/3
  Module3_outputs/4 -> [socParallelAssembly3]
  [socCell3] -> socCellMux/3
  Module3_outputs/3 -> [socCell3]
  [numCyclesCell3] -> numCyclesCellMux/3
  Module3_outputs/2 -> [numCyclesCell3]
  [iCell3] -> iCellMux/3
  Module3_outputs/1 -> [iCell3]
  [vParallelAssembly2] -> vParallelAssemblyMux/2
  Module2_outputs/7 -> [vParallelAssembly2]
  [vCell2] -> vCellMux/2
  Module2_outputs/6 -> [vCell2]
  [temperatureCell2] -> temperatureCellMux/2
  Module2_outputs/5 -> [temperatureCell2]
  [socParallelAssembly2] -> socParallelAssemblyMux/2
  Module2_outputs/4 -> [socParallelAssembly2]
  [socCell2] -> socCellMux/2
  Module2_outputs/3 -> [socCell2]
  [numCyclesCell2] -> numCyclesCellMux/2
  Module2_outputs/2 -> [numCyclesCell2]
  [iCell2] -> iCellMux/2
  Module2_outputs/1 -> [iCell2]
  [vParallelAssembly1] -> vParallelAssemblyMux/1
  vParallelAssemblyMux/1 -> vParallelAssembly/1
  LongModule_outputs/7 -> [vParallelAssembly1]
  [vCell1] -> vCellMux/1
  vCellMux/1 -> vCell/1
  LongModule_outputs/6 -> [vCell1]
  [temperatureCell1] -> temperatureCellMux/1
  temperatureCellMux/1 -> temperatureCell/1
  LongModule_outputs/5 -> [temperatureCell1]
  [socParallelAssembly1] -> socParallelAssemblyMux/1
  socParallelAssemblyMux/1 -> socParallelAssembly/1
  LongModule_outputs/4 -> [socParallelAssembly1]
  [socCell1] -> socCellMux/1
  socCellMux/1 -> socCell/1
  LongModule_outputs/3 -> [socCell1]
  [numCyclesCell1] -> numCyclesCellMux/1
  numCyclesCellMux/1 -> numCyclesCell/1
  LongModule_outputs/2 -> [numCyclesCell1]
  [iCell1] -> iCellMux/1
  iCellMux/1 -> iCell/1
  LongModule_outputs/1 -> [iCell1]
  connections:
  AmbH_To_4/LConn1 -- Module4/LConn1
  AmbH_To_3/LConn1 -- Module3/LConn1
  AmbH_To_2/LConn1 -- Module2/LConn1
  AmbH_From_4/LConn1 -- AmbH/RConn1 -- AmbH_From_3/LConn1 -- AmbH_From_2/LConn1 -- AmbH_From_1/LConn1
  AmbH_To_1/LConn1 -- LongModule/LConn1
  Module4/RConn1 -- -/RConn1
  LongModule/LConn2 -- +/RConn1
  Module4/LConn2 -- Module3/RConn1
  Module3/LConn2 -- Module2/RConn1
  Module2/LConn2 -- LongModule/RConn1
